simulink model "geIAEKF_1x2x2"  (R2023a)
settings: Solver=FixedStepAuto  StartTime=0.0  StopTime=40.0  RelTol=1e-3
values from neighbouring files (symbols this model uses):
  alpha = 0.9999    [Initialization_1x1x1.m]    (also in Initialization_1x2x2.m)
  B = 1    [Initialization_1x1x1.m]    (also in Initialization_1x2x2.m)
  epsilon1 = 0.0000001*eye(K*B)    [Initialization_1x2x2.m]
  fs = 1000    [Initialization_1x1x1.m]    (also in Initialization_1x2x2.m; Initialization_fxKalman.m; Initialization_path_estimation.m)
  K = 1    [Initialization_1x1x1.m]    (also in Initialization_1x2x2.m = 2; Initialization_fxKalman.m = 2)
  m = 4    [Initialization_fxKalman.m]
  N = L*I*J    (= 200)    [Initialization_1x1x1.m]    (also in Initialization_1x2x2.m; Initialization_fxKalman.m = 1)
  P = (5e-6)*eye(N)    [Initialization_1x1x1.m]    (also in Initialization_1x2x2.m; Initialization_fxKalman.m = (5e-6)*eye(M))
  Q = sigma_q^2*eye(N)    [Initialization_1x1x1.m]    (also in Initialization_1x2x2.m)
  Ts = 1/fs    (= 0.001)    [Initialization_1x1x1.m]    (also in Initialization_1x2x2.m; Initialization_fxKalman.m; Initialization_path_estimation.m)
undefined symbols (not defined in the file or in its folder): S11, S12, S21, S22
libraries: simulink x8, speedgoatlib_IO104 x3, matrix_library x2, dspsrcs4 x1
settings Model: Creator=Tamida  LastModifiedBy=tislam
settings SolverCC: ConcurrentTasks=on  PositivePriorityOrder=on
settings OptimizationCC: BlockReduction=off  OptimizeBlockIOStorage=off
settings DebuggingCC: TasksWithSamePriorityMsg=none
settings HardwareCC: ProdBitPerLong=64  ProdLongLongMode=on  ProdHWDeviceType=Intel->x86-64 (Linux 64)
settings RTWCC: Description=Simulink Real-Time  SystemTargetFile=slrealtime.tlc  TemplateMakefile=slrealtime_default_tmf  Toolchain=Simulink Real-Time Toolchain  BuildConfiguration=Faster Runs  CodeExecutionProfiling=on  TargetLang=C++

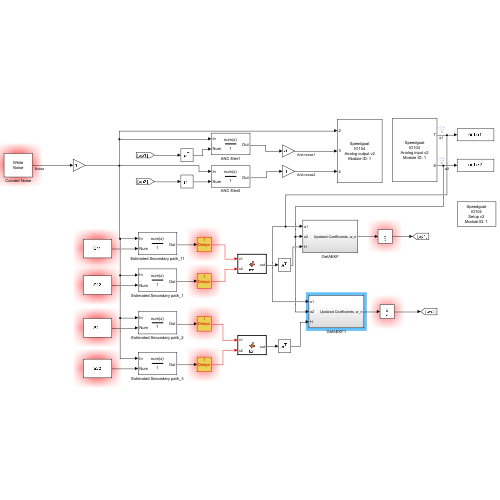
[thumbnail: Simulink's stored preview of the top-level diagram]
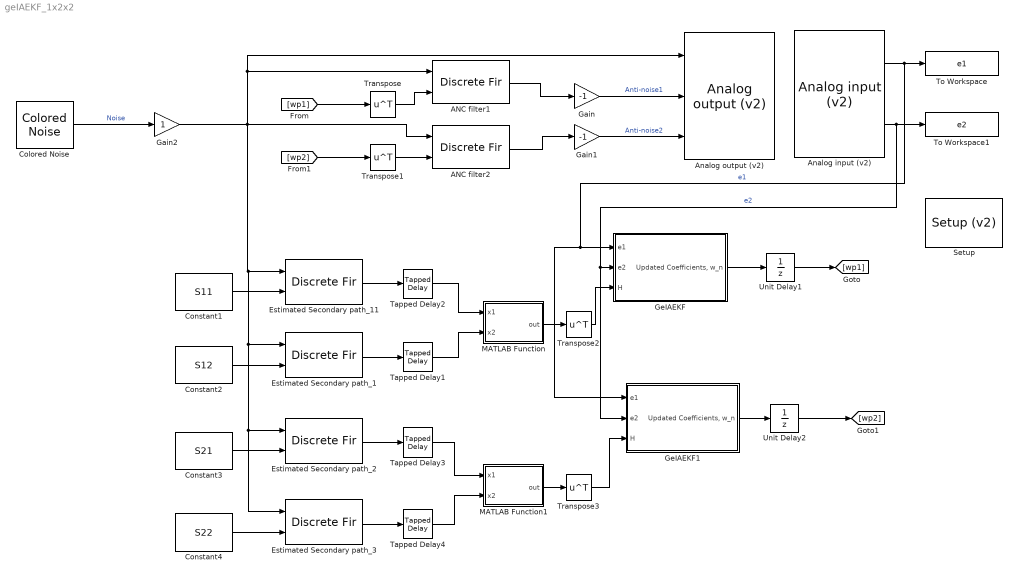
== system geIAEKF_1x2x2 ==
  ANC filter1 : DiscreteFir  CoefSource=Input port
      settings: InputPortMap=u0,u1
  ANC filter2 : DiscreteFir  CoefSource=Input port
      settings: InputPortMap=u0,u1
  "Analog input (v2) " : speedgoatlib_IO104/Analog input (v2)   parModuleId=1  parTs=1/fs  parPciSlot=-1  parAdChannels=[7,8]  parAdChannelsSorted=[7,8]  parAdRange1=+-2.5V  parAdRange2=+-2.5V  parAdCoupling=Differential  parAdFrameSize=1  parAdUseTrigger=off  parAdClockInitiator=Initiator  parAdSampleTime=1.000000000e-03  parTriggerInitiator=Initiator  parTriggerRate=-1.000000000e+00
      settings: SourceProductName=Simulink Real-Time: Speedgoat I/O Blockset
  "Analog output (v2) " : speedgoatlib_IO104/Analog output (v2)   parModuleId=1  parTs=1/fs  parPciSlot=-1  parDaSimultaneous=on  parDaChannels=[2,3,4]  parDaChannelsSorted=[2,3,4]  parDaInitValue=[0,0,0]  parDaReset=[1,1,1]  parDaRange=+-2.5V  parDaFrameSize=1  parDaUseTrigger=off  parDaClockInitiator=Initiator  parDaSampleTime=1.000000000e-03  parTriggerInitiator=Initiator  parTriggerRate=-1.000000000e+00  parAdBlockPresent=1
      settings: SourceProductName=Simulink Real-Time: Speedgoat I/O Blockset
  Colored Noise : dspsrcs4/Colored Noise  Color=white  InverseFrequencyPower=1  BoundedOutput=on  NumChannels=1  OutputDataType=double  SamplesPerFrame=1  SampleTime=Ts  RandomStream=mt19937ar with seed  Seed=67  SimulateUsing=Interpreted execution
      settings: LibrarySourceBlock=audiosources/Colored Noise
  Constant1 : Constant  Value=S11  SampleTime=-1
  Constant2 : Constant  Value=S12  SampleTime=-1
  Constant3 : Constant  Value=S21  SampleTime=-1
  Constant4 : Constant  Value=S22  SampleTime=-1
  Estimated Secondary path_{1..3,11} (4 alike) : DiscreteFir  CoefSource=Input port  Coefficients=[-1.6 -0.6 -.25 0.4 -1.5 0.4 -1.2 0.07 0.6 0.3]
      settings: InputPortMap=u0,u1
  Gain : Gain  Gain=-1
  Gain1 : Gain  Gain=-1
  Gain2 : Gain
  GeIAEKF : Subsystem
  GeIAEKF1 : Subsystem
  MATLAB Function : MATLAB Function  TreatAsAtomicUnit=on
  MATLAB Function1 : MATLAB Function  TreatAsAtomicUnit=on
  Setup : speedgoatlib_IO104/Setup (v2)   parPciSlot=-1  parModuleId=1  parTriggerInitiator=Initiator  parTriggerRate=1/fs  parCalibrate=on  parAdChannels=[7 8]  parAdRange1=+-2.5V  parAdRange2=+-2.5V  parAdCoupling=Differential  parAdUseTrigger=off  parAdFrameSize=1  parAdClockInitiator=Initiator  parAdSampleTime=1/fs  parDaSimultaneous=on  parDaChannels=[2 3 4]  parDaChannelsSorted=[2,3,4]  parDaInitValue=[0]  parDaReset=[1]  parDaRange=+-2.5V  parDaUseTrigger=off  parDaFrameSize=1  parDaClockInitiator=Initiator  parDaSampleTime=1/fs  parDioByte0Dir=Outputs  parDioByte1Dir=Inputs  parDoChannels=0  parDoInitValues=[0]  parDoReset=[1]  parDiChannels=0
      settings: SourceProductName=Simulink Real-Time: Speedgoat I/O Blockset
  Tapped Delay{1..4} (4 alike) : simulink/Discrete/Tapped Delay  vinit=0.0  samptime=-1  NumDelays=(B*N)-1  DelayOrder=Newest  includeCurrent=on
  To Workspace : ToWorkspace  VariableName=e1  SaveFormat=Structure With Time  SampleTime=-1
  To Workspace1 : ToWorkspace  VariableName=e2  SaveFormat=Structure With Time  SampleTime=-1
  Transpose{,1..3} (4 alike) : Math  Operator=transpose
  Unit Delay1 : UnitDelay  SampleTime=Ts  HasFrameUpgradeWarning=on
  Unit Delay2 : UnitDelay  SampleTime=Ts  HasFrameUpgradeWarning=on
  wires:
  Tapped Delay2/1 -> MATLAB Function/1(x1)
  Estimated Secondary path_11/1 -> Tapped Delay2/1
  Constant1/1 -> Estimated Secondary path_11/2
  Transpose2/1 -> GeIAEKF/3(H)
  [wp1] -> Transpose/1
  Transpose/1 -> ANC filter1/2
  ANC filter1/1 -> Gain/1
  GeIAEKF/1("Updated Coefficients, w_n") -> Unit Delay1/1
  Unit Delay1/1 -> [wp1]
  Gain/1 -> "Analog output (v2) "/2  "Anti-noise1"
  "Analog input (v2) "/1 -> GeIAEKF1/1(e1), GeIAEKF/1(e1), To Workspace/1  "e1"
  "Analog input (v2) "/2 -> GeIAEKF1/2(e2), GeIAEKF/2(e2), To Workspace1/1  "e2"
  Constant2/1 -> Estimated Secondary path_1/2
  Estimated Secondary path_1/1 -> Tapped Delay1/1
  Constant3/1 -> Estimated Secondary path_2/2
  Estimated Secondary path_2/1 -> Tapped Delay3/1
  Constant4/1 -> Estimated Secondary path_3/2
  Estimated Secondary path_3/1 -> Tapped Delay4/1
  Gain1/1 -> "Analog output (v2) "/3  "Anti-noise2"
  ANC filter2/1 -> Gain1/1
  Colored Noise/1 -> Gain2/1  "Noise"
  Transpose1/1 -> ANC filter2/2
  [wp2] -> Transpose1/1
  Unit Delay2/1 -> [wp2]
  Tapped Delay1/1 -> MATLAB Function/2(x2)
  Tapped Delay3/1 -> MATLAB Function1/1(x1)
  Tapped Delay4/1 -> MATLAB Function1/2(x2)
  MATLAB Function/1(out) -> Transpose2/1
  MATLAB Function1/1(out) -> Transpose3/1
  GeIAEKF1/1("Updated Coefficients, w_n") -> Unit Delay2/1
  Transpose3/1 -> GeIAEKF1/3(H)
  Gain2/1 -> ANC filter2/1, "Analog output (v2) "/1, ANC filter1/1, Estimated Secondary path_3/1, Estimated Secondary path_2/1, Estimated Secondary path_1/1, Estimated Secondary path_11/1

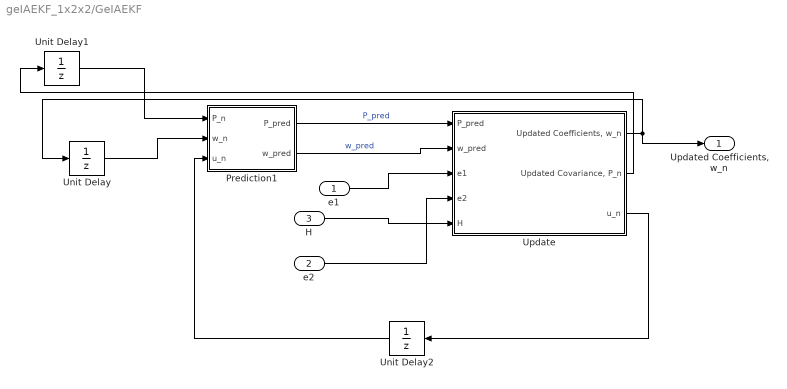
== system geIAEKF_1x2x2/GeIAEKF ==
  e1 : Inport
  e2 : Inport  Port=2
  H : Inport  Port=3
  Prediction1 : Subsystem
  Unit Delay : UnitDelay  InitialCondition=m  SampleTime=Ts  HasFrameUpgradeWarning=on
  Unit Delay1 : UnitDelay  InitialCondition=P  SampleTime=Ts  HasFrameUpgradeWarning=on
  Unit Delay2 : UnitDelay  InitialCondition=m  SampleTime=Ts  HasFrameUpgradeWarning=on
  Update : Subsystem
  "Updated Coefficients, w_n" : Outport
  wires:
  Prediction1/1(P_pred) -> Update/1(P_pred)  "P_pred"
  H/1 -> Update/5(H)
  e1/1 -> Update/3(e1)
  Prediction1/2(w_pred) -> Update/2(w_pred)  "w_pred"
  Update/2("Updated Covariance, P_n") -> Unit Delay1/1
  Update/1("Updated Coefficients, w_n") -> "Updated Coefficients, w_n"/1, Unit Delay/1
  Unit Delay/1 -> Prediction1/2(w_n)
  Unit Delay1/1 -> Prediction1/1(P_n)
  e2/1 -> Update/4(e2)
  Unit Delay2/1 -> Prediction1/3(u_n)
  Update/3(u_n) -> Unit Delay2/1

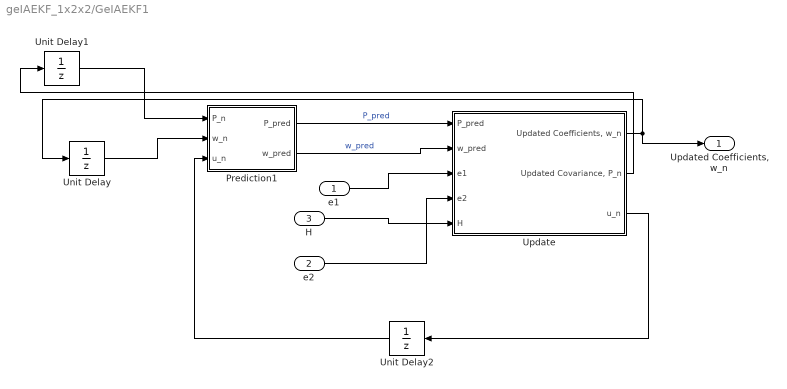
== system geIAEKF_1x2x2/GeIAEKF1 ==
  e1 : Inport
  e2 : Inport  Port=2
  H : Inport  Port=3
  Prediction1 : Subsystem
  Unit Delay : UnitDelay  InitialCondition=m  SampleTime=Ts  HasFrameUpgradeWarning=on
  Unit Delay1 : UnitDelay  InitialCondition=P  SampleTime=Ts  HasFrameUpgradeWarning=on
  Unit Delay2 : UnitDelay  InitialCondition=m  SampleTime=Ts  HasFrameUpgradeWarning=on
  Update : Subsystem
  "Updated Coefficients, w_n" : Outport
  wires:
  Update/3(u_n) -> Unit Delay2/1
  Unit Delay2/1 -> Prediction1/3(u_n)
  e2/1 -> Update/4(e2)
  Unit Delay1/1 -> Prediction1/1(P_n)
  Unit Delay/1 -> Prediction1/2(w_n)
  Update/1("Updated Coefficients, w_n") -> Unit Delay/1, "Updated Coefficients, w_n"/1
  Update/2("Updated Covariance, P_n") -> Unit Delay1/1
  Prediction1/2(w_pred) -> Update/2(w_pred)  "w_pred"
  e1/1 -> Update/3(e1)
  H/1 -> Update/5(H)
  Prediction1/1(P_pred) -> Update/1(P_pred)  "P_pred"

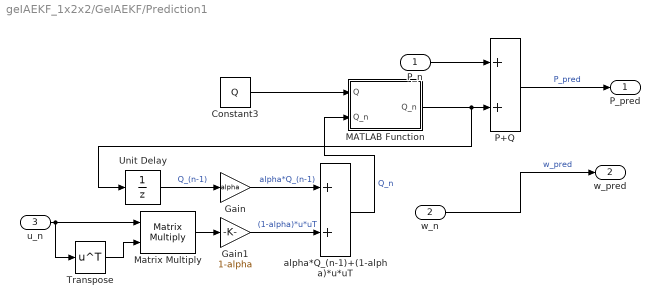
== system geIAEKF_1x2x2/GeIAEKF/Prediction1 ==
  P_n : Inport
  w_n : Inport  Port=2
  u_n : Inport  Port=3
  Constant3 : Constant  Value=Q
  Gain : Gain  Gain=alpha
  Gain1 : Gain  Gain=1-alpha
  MATLAB Function : MATLAB Function  TreatAsAtomicUnit=on
  Matrix Multiply : Product  Multiplication=Matrix(*)
  P+Q : Sum  InputSameDT=on  OutDataTypeStr=Inherit: Inherit via back propagation
  Transpose : Math  Operator=transpose
  Unit Delay : UnitDelay  SampleTime=-1  HasFrameUpgradeWarning=on
  alpha*Q_(n-1)+(1-alpha)*u*uT : Sum  InputSameDT=on  OutDataTypeStr=Inherit: Inherit via back propagation
  P_pred : Outport
  w_pred : Outport  Port=2
  wires:
  P_n/1 -> P+Q/1
  P+Q/1 -> P_pred/1  "P_pred"
  w_n/1 -> w_pred/1  "w_pred"
  MATLAB Function/1(Q_n) -> Unit Delay/1, P+Q/2
  Constant3/1 -> MATLAB Function/1(Q)
  Unit Delay/1 -> Gain/1  "Q_(n-1)"
  Gain/1 -> alpha*Q_(n-1)+(1-alpha)*u*uT/1  "alpha*Q_(n-1)"
  Gain1/1 -> alpha*Q_(n-1)+(1-alpha)*u*uT/2  "(1-alpha)*u*uT"
  alpha*Q_(n-1)+(1-alpha)*u*uT/1 -> MATLAB Function/2("Q_n ")  "Q_n"
  Matrix Multiply/1 -> Gain1/1
  u_n/1 -> Transpose/1, Matrix Multiply/1
  Transpose/1 -> Matrix Multiply/2

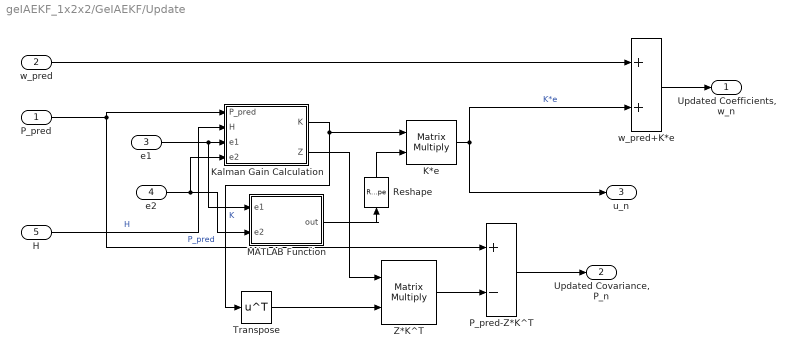
== system geIAEKF_1x2x2/GeIAEKF/Update ==
  P_pred : Inport
  w_pred : Inport  Port=2
  e1 : Inport  Port=3
  e2 : Inport  Port=4
  H : Inport  Port=5
  K*e : Product  Multiplication=Matrix(*)  InputSameDT=on  OutDataTypeStr=Inherit: Inherit via back propagation
  Kalman Gain Calculation : Subsystem
  MATLAB Function : MATLAB Function  TreatAsAtomicUnit=on
  P_pred-Z*K^T : Sum  Inputs=+-  InputSameDT=on  OutDataTypeStr=Inherit: Inherit via back propagation
  Reshape : Reshape  OutputDimensionality=Customize  OutputDimensions=[K*B,1]
  Transpose : Math  Operator=transpose
  Z*K^T : Product  Multiplication=Matrix(*)  InputSameDT=on  OutDataTypeStr=Inherit: Same as first input
  w_pred+K*e : Sum  InputSameDT=on  OutDataTypeStr=Inherit: Inherit via back propagation
  "Updated Coefficients, w_n" : Outport
  "Updated Covariance, P_n" : Outport  Port=2
  u_n : Outport  Port=3
  wires:
  P_pred/1 -> Kalman Gain Calculation/1(P_pred), P_pred-Z*K^T/1  "P_pred"
  Kalman Gain Calculation/1(K) -> Transpose/1, K*e/1  "K"
  Z*K^T/1 -> P_pred-Z*K^T/2
  K*e/1 -> w_pred+K*e/2, u_n/1  "K*e"
  e1/1 -> MATLAB Function/1(e1), Kalman Gain Calculation/3(e1)
  w_pred+K*e/1 -> "Updated Coefficients, w_n"/1
  H/1 -> Kalman Gain Calculation/2(H)  "H"
  w_pred/1 -> w_pred+K*e/1
  P_pred-Z*K^T/1 -> "Updated Covariance, P_n"/1
  Transpose/1 -> Z*K^T/2
  Kalman Gain Calculation/2(Z) -> Z*K^T/1
  e2/1 -> MATLAB Function/2(e2), Kalman Gain Calculation/4(e2)
  MATLAB Function/1(out) -> Reshape/1
  Reshape/1 -> K*e/2

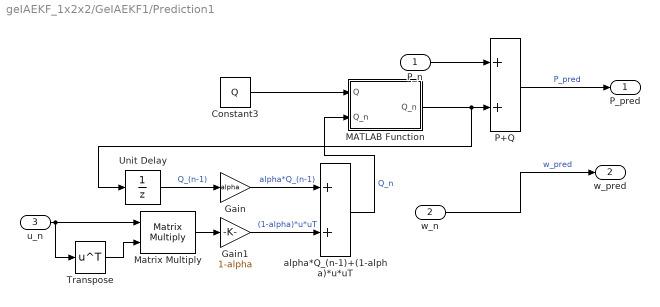
== system geIAEKF_1x2x2/GeIAEKF1/Prediction1 ==
  P_n : Inport
  w_n : Inport  Port=2
  u_n : Inport  Port=3
  Constant3 : Constant  Value=Q
  Gain : Gain  Gain=alpha
  Gain1 : Gain  Gain=1-alpha
  MATLAB Function : MATLAB Function  TreatAsAtomicUnit=on
  Matrix Multiply : Product  Multiplication=Matrix(*)
  P+Q : Sum  InputSameDT=on  OutDataTypeStr=Inherit: Inherit via back propagation
  Transpose : Math  Operator=transpose
  Unit Delay : UnitDelay  SampleTime=-1  HasFrameUpgradeWarning=on
  alpha*Q_(n-1)+(1-alpha)*u*uT : Sum  InputSameDT=on  OutDataTypeStr=Inherit: Inherit via back propagation
  P_pred : Outport
  w_pred : Outport  Port=2
  wires:
  Transpose/1 -> Matrix Multiply/2
  u_n/1 -> Matrix Multiply/1, Transpose/1
  Matrix Multiply/1 -> Gain1/1
  alpha*Q_(n-1)+(1-alpha)*u*uT/1 -> MATLAB Function/2("Q_n ")  "Q_n"
  Gain1/1 -> alpha*Q_(n-1)+(1-alpha)*u*uT/2  "(1-alpha)*u*uT"
  Gain/1 -> alpha*Q_(n-1)+(1-alpha)*u*uT/1  "alpha*Q_(n-1)"
  Unit Delay/1 -> Gain/1  "Q_(n-1)"
  Constant3/1 -> MATLAB Function/1(Q)
  MATLAB Function/1(Q_n) -> P+Q/2, Unit Delay/1
  w_n/1 -> w_pred/1  "w_pred"
  P+Q/1 -> P_pred/1  "P_pred"
  P_n/1 -> P+Q/1

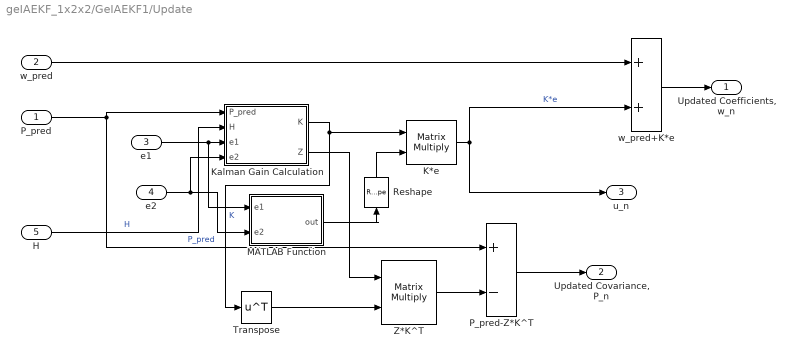
== system geIAEKF_1x2x2/GeIAEKF1/Update ==
  P_pred : Inport
  w_pred : Inport  Port=2
  e1 : Inport  Port=3
  e2 : Inport  Port=4
  H : Inport  Port=5
  K*e : Product  Multiplication=Matrix(*)  InputSameDT=on  OutDataTypeStr=Inherit: Inherit via back propagation
  Kalman Gain Calculation : Subsystem
  MATLAB Function : MATLAB Function  TreatAsAtomicUnit=on
  P_pred-Z*K^T : Sum  Inputs=+-  InputSameDT=on  OutDataTypeStr=Inherit: Inherit via back propagation
  Reshape : Reshape  OutputDimensionality=Customize  OutputDimensions=[K*B,1]
  Transpose : Math  Operator=transpose
  Z*K^T : Product  Multiplication=Matrix(*)  InputSameDT=on  OutDataTypeStr=Inherit: Same as first input
  w_pred+K*e : Sum  InputSameDT=on  OutDataTypeStr=Inherit: Inherit via back propagation
  "Updated Coefficients, w_n" : Outport
  "Updated Covariance, P_n" : Outport  Port=2
  u_n : Outport  Port=3
  wires:
  Reshape/1 -> K*e/2
  MATLAB Function/1(out) -> Reshape/1
  e2/1 -> Kalman Gain Calculation/4(e2), MATLAB Function/2(e2)
  Kalman Gain Calculation/2(Z) -> Z*K^T/1
  Transpose/1 -> Z*K^T/2
  P_pred-Z*K^T/1 -> "Updated Covariance, P_n"/1
  w_pred/1 -> w_pred+K*e/1
  H/1 -> Kalman Gain Calculation/2(H)  "H"
  w_pred+K*e/1 -> "Updated Coefficients, w_n"/1
  e1/1 -> Kalman Gain Calculation/3(e1), MATLAB Function/1(e1)
  K*e/1 -> w_pred+K*e/2, u_n/1  "K*e"
  Z*K^T/1 -> P_pred-Z*K^T/2
  Kalman Gain Calculation/1(K) -> K*e/1, Transpose/1  "K"
  P_pred/1 -> P_pred-Z*K^T/1, Kalman Gain Calculation/1(P_pred)  "P_pred"

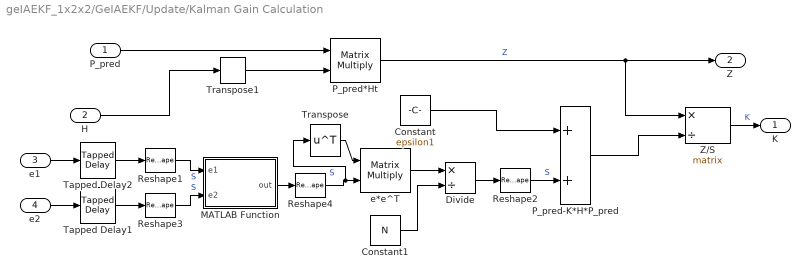
== system geIAEKF_1x2x2/GeIAEKF/Update/Kalman Gain Calculation ==
  P_pred : Inport
  H : Inport  Port=2
  e1 : Inport  Port=3
  e2 : Inport  Port=4
  Constant : Constant  Value=epsilon1  SampleTime=Ts
  Constant1 : Constant  Value=N
  Divide : Product  Inputs=*/
  MATLAB Function : MATLAB Function  TreatAsAtomicUnit=on
  P_pred*Ht : Product  Multiplication=Matrix(*)  InputSameDT=on  OutDataTypeStr=Inherit: Inherit via back propagation
  P_pred-K*H*P_pred : Sum  InputSameDT=on  OutDataTypeStr=Inherit: Inherit via back propagation
  Reshape1 : Reshape  OutputDimensionality=Customize  OutputDimensions=[N,1]
  Reshape2 : Reshape  OutputDimensionality=Customize  OutputDimensions=[K*B,K*B]
  Reshape3 : Reshape  OutputDimensionality=Customize  OutputDimensions=[N,1]
  Reshape4 : Reshape  OutputDimensionality=Customize  OutputDimensions=[N,K*B]
  Tapped Delay1 : simulink/Discrete/Tapped Delay  vinit=0.0  samptime=-1  NumDelays=N-1  DelayOrder=Newest  includeCurrent=on
  Tapped Delay2 : simulink/Discrete/Tapped Delay  vinit=0.0  samptime=-1  NumDelays=N-1  DelayOrder=Newest  includeCurrent=on
  Transpose : Math  Operator=transpose
  Transpose1 : matrix_library/Transpose
  Z/S : Product  Inputs=*/  Multiplication=Matrix(*)
  e*e^T : Product  Multiplication=Matrix(*)  InputSameDT=on  OutDataTypeStr=Inherit: Inherit via back propagation
  K : Outport
  Z : Outport  Port=2
  wires:
  P_pred/1 -> P_pred*Ht/1
  P_pred*Ht/1 -> Z/1, Z/S/1  "Z"
  H/1 -> Transpose1/1
  Transpose1/1 -> P_pred*Ht/2
  Z/S/1 -> K/1  "K"
  e1/1 -> Tapped Delay2/1
  Reshape2/1 -> P_pred-K*H*P_pred/2  "S"
  P_pred-K*H*P_pred/1 -> Z/S/2
  Constant/1 -> P_pred-K*H*P_pred/1
  Tapped Delay2/1 -> Reshape1/1
  Reshape1/1 -> MATLAB Function/1(e1)  "S"
  e*e^T/1 -> Divide/1
  Divide/1 -> Reshape2/1
  Constant1/1 -> Divide/2
  Tapped Delay1/1 -> Reshape3/1
  e2/1 -> Tapped Delay1/1
  Reshape3/1 -> MATLAB Function/2(e2)  "S"
  MATLAB Function/1(out) -> Reshape4/1
  Reshape4/1 -> Transpose/1, e*e^T/2  "S"
  Transpose/1 -> e*e^T/1

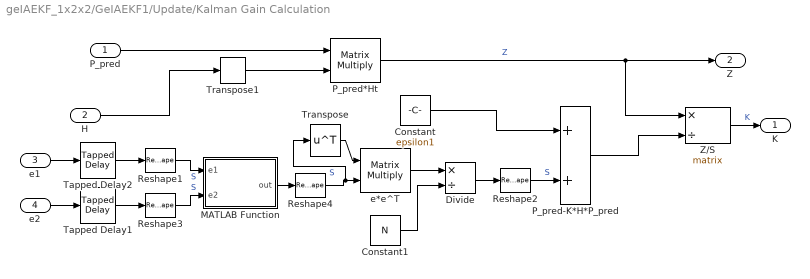
== system geIAEKF_1x2x2/GeIAEKF1/Update/Kalman Gain Calculation ==
  P_pred : Inport
  H : Inport  Port=2
  e1 : Inport  Port=3
  e2 : Inport  Port=4
  Constant : Constant  Value=epsilon1  SampleTime=Ts
  Constant1 : Constant  Value=N
  Divide : Product  Inputs=*/
  MATLAB Function : MATLAB Function  TreatAsAtomicUnit=on
  P_pred*Ht : Product  Multiplication=Matrix(*)  InputSameDT=on  OutDataTypeStr=Inherit: Inherit via back propagation
  P_pred-K*H*P_pred : Sum  InputSameDT=on  OutDataTypeStr=Inherit: Inherit via back propagation
  Reshape1 : Reshape  OutputDimensionality=Customize  OutputDimensions=[N,1]
  Reshape2 : Reshape  OutputDimensionality=Customize  OutputDimensions=[K*B,K*B]
  Reshape3 : Reshape  OutputDimensionality=Customize  OutputDimensions=[N,1]
  Reshape4 : Reshape  OutputDimensionality=Customize  OutputDimensions=[N,K*B]
  Tapped Delay1 : simulink/Discrete/Tapped Delay  vinit=0.0  samptime=-1  NumDelays=N-1  DelayOrder=Newest  includeCurrent=on
  Tapped Delay2 : simulink/Discrete/Tapped Delay  vinit=0.0  samptime=-1  NumDelays=N-1  DelayOrder=Newest  includeCurrent=on
  Transpose : Math  Operator=transpose
  Transpose1 : matrix_library/Transpose
  Z/S : Product  Inputs=*/  Multiplication=Matrix(*)
  e*e^T : Product  Multiplication=Matrix(*)  InputSameDT=on  OutDataTypeStr=Inherit: Inherit via back propagation
  K : Outport
  Z : Outport  Port=2
  wires:
  Transpose/1 -> e*e^T/1
  Reshape4/1 -> e*e^T/2, Transpose/1  "S"
  MATLAB Function/1(out) -> Reshape4/1
  Reshape3/1 -> MATLAB Function/2(e2)  "S"
  e2/1 -> Tapped Delay1/1
  Tapped Delay1/1 -> Reshape3/1
  Constant1/1 -> Divide/2
  Divide/1 -> Reshape2/1
  e*e^T/1 -> Divide/1
  Reshape1/1 -> MATLAB Function/1(e1)  "S"
  Tapped Delay2/1 -> Reshape1/1
  Constant/1 -> P_pred-K*H*P_pred/1
  P_pred-K*H*P_pred/1 -> Z/S/2
  Reshape2/1 -> P_pred-K*H*P_pred/2  "S"
  e1/1 -> Tapped Delay2/1
  Z/S/1 -> K/1  "K"
  Transpose1/1 -> P_pred*Ht/2
  H/1 -> Transpose1/1
  P_pred*Ht/1 -> Z/S/1, Z/1  "Z"
  P_pred/1 -> P_pred*Ht/1

== matlab function geIAEKF_1x2x2/MATLAB Function ==
  data: x1 input; out output; x2 input
function out = fcn(x1, x2)

%#codegen

out = [x1, x2]; % 200x2 matrix

== matlab function geIAEKF_1x2x2/GeIAEKF1/Prediction1/MATLAB Function ==
  data: Q input; Q_n output; Q_n input
function Q_n = fcn(Q, Q_n)

%#codegen
if Q_n<Q
    Q_n = Q; 
else
    Q_n = Q_n;
end

== matlab function geIAEKF_1x2x2/GeIAEKF1/Update/Kalman Gain Calculation/MATLAB Function ==
  data: e1 input; out output; e2 input
function out = fcn(e1, e2)

%#codegen

out = [e1, e2]; % 200x2 matrix

== matlab function geIAEKF_1x2x2/GeIAEKF1/Update/MATLAB Function ==
  data: e1 input; out output; e2 input
function out = fcn(e1, e2)

%#codegen

out = [e1, e2]; % 200x2 matrix

== matlab function geIAEKF_1x2x2/GeIAEKF/Update/Kalman Gain Calculation/MATLAB Function ==
  data: e1 input; out output; e2 input
function out = fcn(e1, e2)

%#codegen

out = [e1, e2]; % 200x2 matrix

== matlab function geIAEKF_1x2x2/GeIAEKF/Update/MATLAB Function ==
  data: e1 input; out output; e2 input
function out = fcn(e1, e2)

%#codegen

out = [e1, e2]; % 200x2 matrix

== matlab function geIAEKF_1x2x2/GeIAEKF/Prediction1/MATLAB Function ==
  data: Q input; Q_n output; Q_n input
function Q_n = fcn(Q, Q_n)

%#codegen
if Q_n<Q
    Q_n = Q; 
else
    Q_n = Q_n;
end

== matlab function geIAEKF_1x2x2/MATLAB Function1 ==
  data: x1 input; out output; x2 input
function out = fcn(x1, x2)

%#codegen

out = [x1, x2]; % 200x2 matrix
